simulink model "ex_rotor_bars_motor"  (R2026b)
settings: Solver=ode23t  StopTime=2  MaxStep=1e-4  RelTol=1e-5
undefined symbols (not defined in the file or in its folder): L1, L2, L3, Rechtsdrehfeld
libraries: asm_blocks_lib x16, nesl_utility x1
settings Model: Creator=fsbb  LastModifiedBy=fsbb
settings SimscapeCC: SimscapeLogType=all  SimscapeNominalValues="[{\"value\":\"1\",\"unit\":\"A\"},{\"value\":\"1\",\"unit\":\"bar\"},{\"value\":\"1\",\"unit\":\"cm^2\"},{\"value\":\"1\",\"unit\":\"cm^3/s\"},{\"value\":\"1\",\"unit\":\"kJ/kg\"},{\"value\":\"1\",\"unit\":\"kW\"},{\"value\":\"1\",\"unit\":\"l\"},{\"value\":\"1\",\"unit\":\"N\"},{\"value\":\"1\",\"unit\":\"N*m\"},{\"value\":\"1\",\"unit\":\"V\"},{\"value\":\"0.001\",\"unit\":\"Wb\"}]"  SimscapeUseEnergyAccounting=off

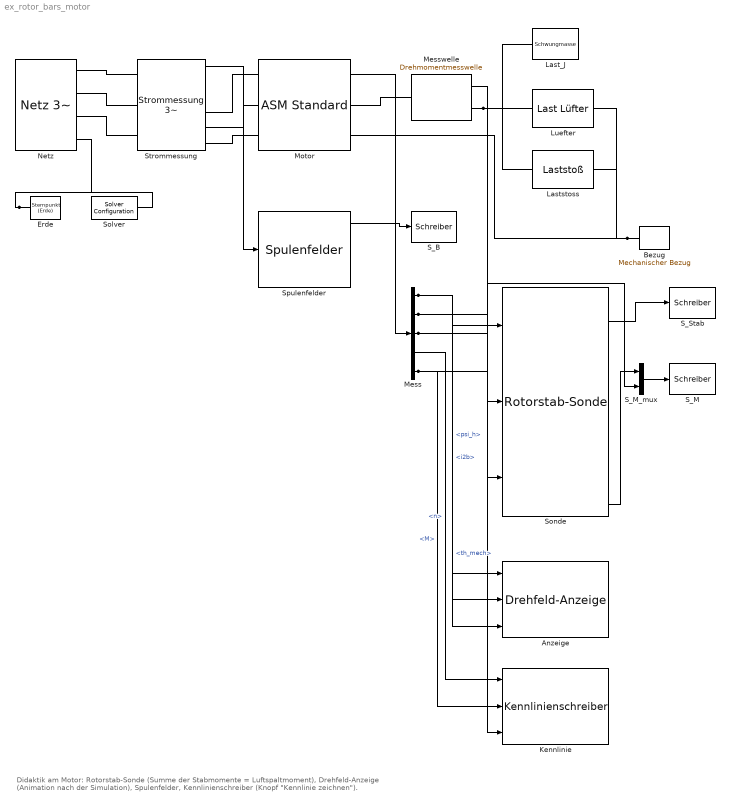
== system ex_rotor_bars_motor ==
  note: Didaktik am Motor: Rotorstab-Sonde (Summe der Stabmomente = Luftspaltmoment), Drehfeld-Anzeige (Animation nach der Simulation), Spulenfelder, Kennlinienschreiber (Knopf "Kennlinie zeichnen").
  Anzeige : asm_blocks_lib/Didaktik/Drehfeld-Anzeige  Tag=asmlib:field_display  view_frame=statorfest  image_orientation=wie Folien (U1 oben, Feld im Uhrzeigersinn)  decomposition=on  change_vector=on  force_arrows=on  all_bars=on  slow_motion=0.05  N2=28  p=2  l=0.15  r=0.06  N1xi1=144  bar1_angle=-90
  Bezug : asm_blocks_lib/Mechanik/Mechanischer Bezug  Tag=asmlib:mech_reference
  Erde : asm_blocks_lib/Quellen/Sternpunkt (Erde)  Tag=asmlib:neutral_ground
  Kennlinie : asm_blocks_lib/Didaktik/Kennlinienschreiber  Tag=asmlib:torque_speed_recorder  show_kloss=on  show_ec=on  MK=71.55  sK=0.2  ns=1500
  Last_J : asm_blocks_lib/Mechanik/Schwungmasse  Tag=asmlib:inertia  J=0.01  n0=0
  Laststoss : asm_blocks_lib/Mechanik/Laststoß  Tag=asmlib:load_step  t_step=1  dM_L=7.95
  Luefter : asm_blocks_lib/Mechanik/Last Lüfter  Tag=asmlib:load_fan  M_B=26.5  n_B=1440
  Mess : BusSelector  OutputSignals=psi_h,i2b,th_mech,n,M
  Messwelle : asm_blocks_lib/Messgeräte/Drehmomentmesswelle  Tag=asmlib:torque_sensor
  Motor : asm_blocks_lib/Maschine/ASM Standard  Tag=asmlib:asm_standard  param_set=Standard  connection=Stern  U_N=400  f_N=50  p=2  R1=0.5  L1s=0.009902  Lh=0.25  R2b=1.225  L2sb=0.009902  J_M=0.012  k_R=0  n0=0  l=0.15  r=0.06  N2=28  Bhat_N=0.8
  Netz : asm_blocks_lib/Quellen/Netz 3~  Tag=asmlib:grid3  U_L=400  f1=50  phase_seq=L1-L2-L3 (Rechtsdrehfeld)  phi0=0  t_on=0  R_N=0  L_N=0
  S_B : asm_blocks_lib/Messgeräte/Schreiber  Tag=asmlib:recorder  title_text=Spulenfelder B_U, B_V, B_W
  S_M : asm_blocks_lib/Messgeräte/Schreiber  Tag=asmlib:recorder  title_text=Summe der Stabmomente und Luftspaltmoment
  S_M_mux : Mux  Inputs=2
  S_Stab : asm_blocks_lib/Messgeräte/Schreiber  Tag=asmlib:recorder  title_text=Strom Stab 1 und 2
  Solver : nesl_utility/Solver Configuration  PhysicalDomain=network_engine_domain  SubClassName=solver  LeftPortType=input  RightPortType=generic  Tones=[]  Harmonics=[]  SimulateNoise=off  Profile=off  UseLocalSampling=off  EnableSwitchedLinearOptims=on  FrequencyDomain=off  UseCCode=off  RelTol=0.001  AbsTol=0.001  MinStep=1e-09  ToWorkspace=off  RevertToSquareIcSolve=off  NumHomotopyIterations=100  PhasorMode=off  PhasorModeNumHarmonics=1  ConsistencySolver=NEWTON_XTOL_AFTER_FTOL  CanonicalOrdering=CANONICAL  OptimizeIntermediates=OPTIMIZED  MulticoreSolverChoice=BACKWARD_EULER  IndexReductionMethod=DerivativeReplacement  DoDC=off  ResidualTolerance=1e-09  ConsistencyTolSource=GLOBAL  ConsistencyAbsTol=0.001  ConsistencyRelTol=0.001  ConsistencyTolFactor=0.001  UseLocalSolver=off  LocalSolverChoice=NE_BACKWARD_EULER_ADVANCER  ResolveIndetEquations=on  FunctionEvalNumThread=1  LocalSolverSampleTime=0.001  DoFixedCost=off  MaxNonlinIter=3  MaxModeIter=2  ComputeImpulses=off  ImpulseIterations=2  LinearAlgebra=auto  LinearAlgebraNumThread=0  EquationFormulation=NE_TIME_EF  DelaysMemoryBudget=1024  AutomaticFiltering=on  FilteringTimeConstant=0.001  PartitionStorageMethod=AS_NEEDED  PartitionMemoryBudget=1024  PartitionMethod=BALANCED  MultibodyUseLocalSolver=off  MultibodyLocalSolverChoice=ODE1  MultibodyLocalSolverSampleTime=0.001
  Sonde : asm_blocks_lib/Didaktik/Rotorstab-Sonde  Tag=asmlib:rotor_bar_probe  k1=1  k2=8  N2=28  p=2  l=0.15  r=0.06  N1xi1=144  bar1_angle=-90  convention=wie Folien (Strom aus der Zeichenebene positiv)
  Spulenfelder : asm_blocks_lib/Didaktik/Spulenfelder  Tag=asmlib:coil_fields  Lh=0.25  N1xi1=144  p=2  l=0.15  r=0.06
  Strommessung : asm_blocks_lib/Messgeräte/Strommessung 3~  Tag=asmlib:current_sensor3  f_meas=50
  wires:
  Motor/1 -> Mess/1
  Mess/1 -> Sonde/1, Anzeige/1  "<psi_h>"
  Mess/2 -> Sonde/2, Anzeige/2  "<i2b>"
  Mess/3 -> Sonde/3, Anzeige/3  "<th_mech>"
  Mess/4 -> Kennlinie/1  "<n>"
  Mess/5 -> Kennlinie/2, S_M_mux/2  "<M>"
  Messwelle/1 -> Kennlinie/3
  Strommessung/1 -> Spulenfelder/1
  Sonde/2 -> S_Stab/1
  Sonde/10 -> S_M_mux/1
  S_M_mux/1 -> S_M/1
  Spulenfelder/1 -> S_B/1
  connections:
  Erde/LConn1 -- Netz/RConn4 -- Solver/RConn1
  Netz/RConn1 -- Strommessung/LConn1
  Strommessung/RConn1 -- Motor/LConn1
  Netz/RConn2 -- Strommessung/LConn2
  Strommessung/RConn2 -- Motor/LConn2
  Netz/RConn3 -- Strommessung/LConn3
  Strommessung/RConn3 -- Motor/LConn3
  Motor/RConn1 -- Messwelle/LConn1
  Motor/RConn2 -- Luefter/RConn1 -- Bezug/LConn1 -- Laststoss/RConn1
  Last_J/LConn1 -- Messwelle/RConn1 -- Luefter/LConn1 -- Laststoss/LConn1
